simulink subsystem "removeZero"  (R2026a)
settings: Solver=VariableStepAuto
settings Model: Creator=maxhu  LastModifiedBy=maxhu

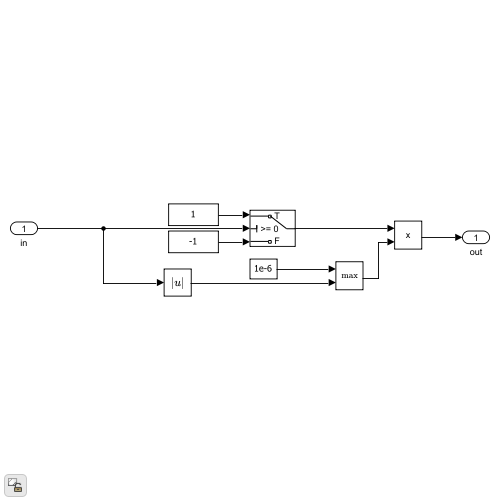
[thumbnail: Simulink's stored preview of the top-level diagram]
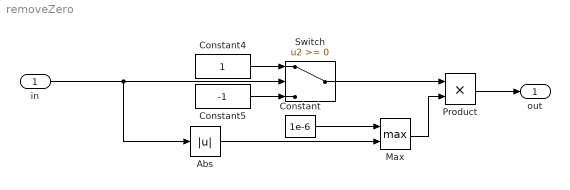
== system removeZero ==
  in : Inport
  Abs : Abs  SaturateOnIntegerOverflow=off
  Constant : Constant  Value=1e-6
  Constant4 : Constant
  Constant5 : Constant  Value=-1
  Max : MinMax  Function=max  Inputs=2
  Product : Product
  Switch : Switch  SaturateOnIntegerOverflow=off  InputSameDT=off
  out : Outport
  wires:
  Switch/1 -> Product/1
  Product/1 -> out/1
  Max/1 -> Product/2
  Constant/1 -> Max/1
  Constant5/1 -> Switch/3
  Constant4/1 -> Switch/1
  in/1 -> Abs/1, Switch/2
  Abs/1 -> Max/2
